simulink model "IEEE39_AvgInverter_Native"  (R2025a)
settings: Solver=ode4  StartTime=0.0  StopTime=0.20000000000000001  FixedStep=1e-6  RelTol=1e-3
settings Model: Creator=matthiasmees  LastModifiedBy=matthiasmees
settings DataIOCC: ExternalInput=vabc  LoadExternalInput=on

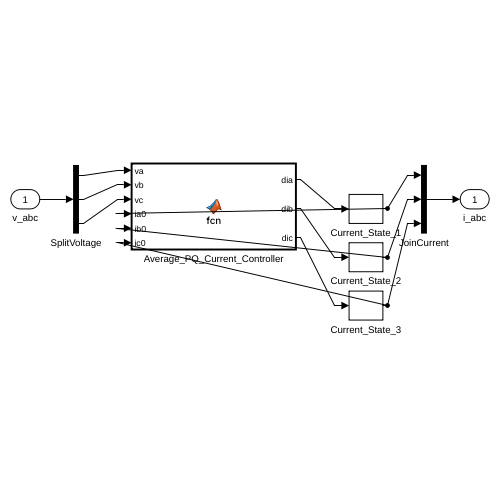
[thumbnail: Simulink's stored preview of the top-level diagram]
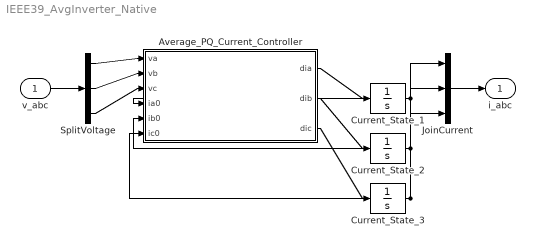
== system IEEE39_AvgInverter_Native ==
  v_abc : Inport  PortDimensions=3
  Average_PQ_Current_Controller : MATLAB Function  TreatAsAtomicUnit=on
  Current_State_1 : Integrator
  Current_State_2 : Integrator
  Current_State_3 : Integrator
  JoinCurrent : Mux  Inputs=3
  SplitVoltage : Demux  Outputs=3
  i_abc : Outport  PortDimensions=3
  wires:
  v_abc/1 -> SplitVoltage/1
  SplitVoltage/1 -> Average_PQ_Current_Controller/1(va)
  Current_State_1/1 -> Average_PQ_Current_Controller/4(ia0), JoinCurrent/1
  Average_PQ_Current_Controller/1(dia) -> Current_State_1/1
  SplitVoltage/2 -> Average_PQ_Current_Controller/2(vb)
  Current_State_2/1 -> Average_PQ_Current_Controller/5(ib0), JoinCurrent/2
  Average_PQ_Current_Controller/2(dib) -> Current_State_2/1
  SplitVoltage/3 -> Average_PQ_Current_Controller/3(vc)
  Current_State_3/1 -> Average_PQ_Current_Controller/6(ic0), JoinCurrent/3
  Average_PQ_Current_Controller/3(dic) -> Current_State_3/1
  JoinCurrent/1 -> i_abc/1

== matlab function IEEE39_AvgInverter_Native/Average_PQ_Current_Controller ==
  data: va input; dia output; vb input; vc input; ia0 input; ib0 input; ic0 input; dib output; dic output
function [dia,dib,dic] = fcn(va,vb,vc,ia0,ib0,ic0)
%#codegen
P = 250e6; Q = 161.762e6; Vnom = 25e3; Ipu = 1.20; tau = 5e-3;
a = (2/3)*(va-0.5*vb-0.5*vc);
b = (2/3)*(sqrt(3)/2)*(vb-vc);
v2 = a*a + b*b;
if v2 < 1, iaref = 0; ibref = 0; icref = 0;
else
  k = 2/(3*v2);
  ialpha = k*(P*a + Q*b); ibeta = k*(P*b-Q*a);
  imax = Ipu*sqrt(2)*hypot(P,Q)/(sqrt(3)*Vnom);
  imag = hypot(ialpha,ibeta);
  if imag > imax, ialpha=ialpha*imax/imag; ibeta=ibeta*imax/imag; end
  iaref = ialpha; ibref = -0.5*ialpha+sqrt(3)/2*ibeta;
  icref = -0.5*ialpha-sqrt(3)/2*ibeta;
end
dia=(-iaref-ia0)/tau; dib=(-ibref-ib0)/tau; dic=(-icref-ic0)/tau;
end
